simulink model "QD2_Sim_Dual"  (R2023b)
settings: Solver=FixedStepDiscrete  StartTime=0.0  StopTime=400  FixedStep=0.002  RelTol=1e-3
PreLoadFcn:
  | % QD2_Sim_Dual: agrega lib/ y sim/ al path antes de cargar (enlaces a QD2_Mission_Lib)
  | qd2_c = {pwd};
  | qd2_w = which('QD2_Sim_Dual');
  | if ~isempty(qd2_w), qd2_c{end+1} = fileparts(qd2_w); end
  | for qd2_i = 1:numel(qd2_c)
  |     qd2_d = qd2_c{qd2_i};
  |     for qd2_k = 1:4
  |         if exist(fullfile(qd2_d, 'lib', 'QD2_Mission_Lib.slx'), 'file')
  |             addpath(fullfile(qd2_d, 'lib'));
  |             addpath(fullfile(qd2_d, 'sim'));
  |             break;
  |         end
  |         qd2_d = fileparts(qd2_d);
  |     end
  | end
  | clear qd2_c qd2_w qd2_i qd2_d qd2_k
PostLoadFcn:
  | % QD2_Sim_Dual: rutas de lib/ (funciones qd2_* y QD2_Mission_Lib) y sim/
  | qd2_d = fileparts(get_param(bdroot, 'FileName'));
  | for qd2_k = 1:4
  |     if exist(fullfile(qd2_d, 'lib', 'qd2_params.m'), 'file'), break; end
  |     qd2_d = fileparts(qd2_d);
  | end
  | addpath(fullfile(qd2_d, 'lib'));
  | addpath(fullfile(qd2_d, 'sim'));
  | clear qd2_d qd2_k
InitFcn:
  | % QD2_Sim_Dual: rutas de lib/ (funciones qd2_* y QD2_Mission_Lib) y sim/
  | qd2_d = fileparts(get_param(bdroot, 'FileName'));
  | for qd2_k = 1:4
  |     if exist(fullfile(qd2_d, 'lib', 'qd2_params.m'), 'file'), break; end
  |     qd2_d = fileparts(qd2_d);
  | end
  | addpath(fullfile(qd2_d, 'lib'));
  | addpath(fullfile(qd2_d, 'sim'));
  | clear qd2_d qd2_k
  | % Parámetros (config/estacion.json es la única fuente de verdad)
  | QD2P = qd2_params_from_config();
  | QD2_SIM = qd2_sim_parametros();
  | % La versión la fija el bloque constante VERSION de la raíz
  | QD2_VERSION = str2double(get_param([bdroot '/' sprintf('VERSION\n(1 = PID, 2 = MPC)')], 'Value'));
libraries: simulink x1
(part 2 of 2)

== matlab function QD2_Sim_Dual/MISSION SUPERVISOR/MATLAB Function ==
  data: t input; sp1 output size=[4 1]; pose1 input; pose2 input; trk input; py input; ab input; sp2 output size=[4 1]; ctx output size=[7 1]; info output size=[40 1]; estado output size=1; cmd1 output size=[3 1]; cmd2 output size=[3 1]; P parameter; version parameter
function [sp1, sp2, ctx, info, estado, cmd1, cmd2] = fcn(t, pose1, pose2, trk, py, ab, P, version)
%#codegen
% MISSION SUPERVISOR: qd2_mission_step (FSM de ARQUITECTURA §3.3) para los 2 drones.
% ab = Onboard Status [fsm1 fsm2 cod1 cod2] (MPC LINK CHECK; fsm 0 = desconocida;
% cod 0 bien, 1 protocolo MPC incorrecto, 2 enlace perdido).
persistent s
if isempty(s)
    s = qd2_mission_init(P);
end
in.t = t;
in.pose1 = [pose1(1) pose1(2) pose1(3) pose1(4)];
in.pose2 = [pose2(1) pose2(2) pose2(3) pose2(4)];
in.tracked1 = trk(1);
in.tracked2 = trk(2);
in.py = py(:);
in.version = version;
in.fsm_a_bordo = [ab(1) ab(2)];
in.proto_mal = [ab(3) ab(4)];
[s, ~, ~, tel] = qd2_mission_step(s, in, P);
sp1 = [tel.sp1(1); tel.sp1(2); tel.sp1(3); tel.sp1(4)];
sp2 = [tel.sp2(1); tel.sp2(2); tel.sp2(3); tel.sp2(4)];
cmd1 = [tel.arm(1); tel.takeoff(1); tel.estop(1)];
cmd2 = [tel.arm(2); tel.takeoff(2); tel.estop(2)];
ctx = zeros(7, 1);
ctx(1) = tel.explorer_id;
for k = 1:6
    ctx(k+1) = tel.ctx_guard(k);
end
% Mission Info [40] (orden fijo, lo leen el TELEMETRY PACK, el OPERATOR SAFETY LAYER
% (info(1)) y el SETPOINT RATE LIMITER (info(38:39)))
info = zeros(40, 1);
info(1) = tel.mission_state;      info(2) = tel.explorer_id;
info(3) = tel.responder_id;       info(4) = tel.explorer_wp_idx;
info(5) = tel.explorer_wp_total;  info(6) = tel.responder_target_id;
info(7) = tel.n_targets_known;    info(8) = tel.n_targets_visited;
info(9) = tel.explorer_done;      info(10) = tel.visited_mask;
info(11) = tel.marking_progress;  info(12) = tel.queue_length;
info(13) = tel.cmd_seq_ack;
info(14) = tel.home1(1);  info(15) = tel.home1(2);
info(16) = tel.home2(1);  info(17) = tel.home2(2);
info(18) = tel.role1;     info(19) = tel.role2;
info(20) = tel.alerta;    info(21) = tel.home_ok;
info(22) = tel.pausa_por_trk;  info(23) = tel.hb_ok;
info(24) = tel.pausa_por_hb;   info(25) = tel.z_E;
info(26) = tel.z_R;       info(27) = tel.d_min_h;
info(28) = tel.t_mark;    info(29) = tel.r_marking;
% falla a bordo por dron (0, 9, 10), fase de la reacción, objetivo rotando y(56:60)
info(30) = tel.falla(1);  info(31) = tel.falla(2);
info(32) = tel.falla_fase;
for k = 1:5
    info(32 + k) = tel.obj_rot(k);
end
% 1 = el dron se aparta de un dron en falla (límite xy P.falla_rate_xy)
info(38) = tel.escape(1); info(39) = tel.escape(2);
estado = tel.mission_state;

== matlab function QD2_Sim_Dual/MPC LINK CHECK/MATLAB Function ==
  data: t input; est output size=[4 1]; tel1 input; tel2 input; lb1 input; lb2 input; cs1 input; cs2 input; P parameter; version parameter
function est = fcn(t, tel1, tel2, lb1, lb2, cs1, cs2, P, version)
%#codegen
% MPC LINK CHECK (qd2_enlace_mpc): valida la respuesta de 8 doubles de cada dron
% (§3.2: y(8) = 2, FSM entera 1..9). est = [fsm1 fsm2 cod1 cod2]
% (cod 0 bien, 1 protocolo incorrecto sostenido, 2 enlace perdido).
persistent tm
if isempty(tm)
    tm = [-1 -1 0 0];
end
y1 = zeros(1, 8);
y2 = zeros(1, 8);
for k = 1:8
    y1(k) = tel1(k);
    y2(k) = tel2(k);
end
[e, tm] = qd2_enlace_mpc(tm, t, y1, y2, [lb1(1) lb2(1)], [cs1(1) cs2(1)], P, version);
est = [e(1); e(2); e(3); e(4)];

== matlab function QD2_Sim_Dual/QDRONE 2 #1 (SIM)/PLANT (qd2_quad_plant) ==
  data: u input; x output size=[10 1]; F input; home input; QD2P parameter
function x = fcn(u, F, home, QD2P)
%#codegen
% PLANTA: qd2_quad_plant (traslación 3D, actitud y empuje de 1er orden, suelo).
persistent xs
if isempty(xs)
    xs = zeros(10, 1);
    xs(1) = home(1);
    xs(2) = home(2);
end
xs = qd2_quad_plant(xs, u, F, 0.002, QD2P.planta);
x = xs;

== matlab function QD2_Sim_Dual/OPERATOR SAFETY LAYER/MATLAB Function ==
  data: t input; trig1 output size=[1 4]; sw input; cmd1 input; cmd2 input; modo_sel input; trig2 output size=[1 4]; modo_ef output size=1
function [trig1, trig2, modo_ef] = fcn(t, sw, cmd1, cmd2, modo_sel)
%#codegen
% OPERATOR SAFETY LAYER (versión simple, interfaz de la simulación QD2_Sim_Dual).
% sw = [Arm Takeoff EStop 0]. modo 0 = MISIÓN, 1 = MANUAL Equipo2 (solo dron 1).
EXT = false;
D_MIN = 0.9;
estado = -1;
fsm = [0 0];
d1 = zeros(7, 1);
d2 = zeros(7, 1);
T_ARM_MIN = 1.0;    % s armado antes de permitir takeoff (a bordo: trigger_2 en IDLE = Error)
T_ACEPTA = 2.0;     % s para que el supervisor acepte el LAND ALL del operador
T_RESPALDO = 90.0;  % s máximos con Takeoff/Land abajo antes del aterrizaje crudo
Z_SUELO = 0.10;     % m
persistent modo t_arm a_prev to_prev sw_prev t_bajo n_req lat_to lat_arm
if isempty(modo)
    modo = double(modo_sel > 0.5);
    t_arm = [-1 -1];
    a_prev = [0 0];
    to_prev = [0 0];
    sw_prev = [double(sw(1) > 0.5) double(sw(2) > 0.5) double(sw(3) > 0.5)];
    t_bajo = -1;
    n_req = 0;
    lat_to = 0;
    lat_arm = 0;
end
sw_arm = sw(1) > 0.5;
sw_to = sw(2) > 0.5;
sw_es = sw(3) > 0.5;
z = [d1(3) d2(3)];
rastreo = [d1(7) > 0.5 && isfinite(d1(3)), d2(7) > 0.5 && isfinite(d2(3))];
armado = a_prev(1) > 0.5 || a_prev(2) > 0.5;
volando = to_prev(1) > 0.5 || to_prev(2) > 0.5;

% ---- Cambio de modo: SOLO en tierra, con los dos Flight State en Idle (0),
% los dos desarmados y los switches Arm y Takeoff ABAJO. Así un cambio del
% selector hecho en vuelo queda pendiente y nunca dispara arm/takeoff solo:
% el operador tiene que bajar los switches y volver a subirlos.
sel = double(modo_sel > 0.5);
suelo = true;
for i = 1:2
    if rastreo(i) && z(i) >= Z_SUELO
        suelo = false;
    end
end
if sel ~= modo && fsm(1) == 0 && fsm(2) == 0 && ~armado && ~volando && ~sw_arm && ~sw_to && suelo
    modo = sel;
    t_arm = [-1 -1];
end

% ---- Peticiones del operador en modo MISIÓN (flancos de los switches)
if EXT && modo < 0.5
    if sw_prev(2) > 0.5 && ~sw_to && (armado || volando)
        n_req = n_req + 1;      % Takeoff/Land abajo -> LAND ALL ordenado
        lat_to = 1;
        t_bajo = t;
    end
    if sw_prev(1) > 0.5 && ~sw_arm && armado
        n_req = n_req + 1;      % Arm abajo (corte, como el original) -> LAND ALL
        lat_arm = 1;
    end
    if sw_prev(3) < 0.5 && sw_es && armado
        n_req = n_req + 1;      % E-stop -> LAND ALL (la misión no sigue)
    end
end
if sw_to
    lat_to = 0;
    t_bajo = -1;
end
if sw_arm
    lat_arm = 0;
end
sw_prev = [double(sw_arm) double(sw_to) double(sw_es)];

% ---- Disparos pedidos
if modo > 0.5
    a = [double(sw_arm) 0];
    to_req = [sw_to false];
    es = [double(sw_es) double(sw_es)];
else
    a = [double(sw_arm && cmd1(1) > 0.5), double(sw_arm && cmd2(1) > 0.5)];
    es = [double(sw_es || cmd1(3) > 0.5), double(sw_es || cmd2(3) > 0.5)];
    if EXT
        % Takeoff/Land = PERMISO para despegar. En vuelo, bajarlo NO corta el
        % takeoff de golpe (cada dron aterrizaría en su x,y: E caería sobre R
        % en la versión MPC); pide LAND ALL y el takeoff sigue al supervisor.
        to_req = [cmd1(2) > 0.5 && (sw_to || to_prev(1) > 0.5), ...
                  cmd2(2) > 0.5 && (sw_to || to_prev(2) > 0.5)];
    else
        to_req = [sw_to && cmd1(2) > 0.5, sw_to && cmd2(2) > 0.5];
    end
end

% ---- Respaldo crudo: el supervisor no aceptó el LAND ALL (estado distinto de
% LANDING/DONE/en tierra) en T_ACEPTA, o pasaron T_RESPALDO con Takeoff abajo.
% Suelta el takeoff, pero NUNCA el de un dron que tiene al otro DEBAJO a
% menos de d_min_h en horizontal (aterrizaría encima / en su downwash).
respaldo = 0;
if EXT && modo < 0.5 && t_bajo >= 0 && volando
    acepto = (estado == 7) || (estado == 8) || (estado <= 2);
    if (~acepto && (t - t_bajo) >= T_ACEPTA) || ((t - t_bajo) >= T_RESPALDO)
        respaldo = 1;
        dh = sqrt((d1(1) - d2(1))^2 + (d1(2) - d2(2))^2);
        for i = 1:2
            o = 3 - i;
            debajo = rastreo(o) && rastreo(i) && dh < D_MIN && z(o) < z(i) - 0.15;
            if ~debajo
                to_req(i) = false;
            end
        end
    end
end

% ---- Takeoff efectivo: >= T_ARM_MIN después de armar (también en MANUAL).
to = [0 0];
for i = 1:2
    if a(i) > 0.5
        if t_arm(i) < 0
            t_arm(i) = t;
        end
    else
        t_arm(i) = -1;
    end
    if modo > 0.5
        % manual: igual que el original una vez en vuelo (el takeoff sigue al
        % switch aunque se baje Arm); para despegar exige 1 s armado
        if to_req(i) && (to_prev(i) > 0.5 || (a(i) > 0.5 && (t - t_arm(i)) >= T_ARM_MIN))
            to(i) = 1;
        end
    elseif to_req(i) && a(i) > 0.5 && (t - t_arm(i)) >= T_ARM_MIN
        to(i) = 1;
    end
end

% ---- Alerta del operador para la telemetría (y(55))
codigo = 0;
if sw_es
    codigo = 5;
elseif respaldo > 0.5
    codigo = 8;
elseif lat_arm > 0.5
    codigo = 7;
elseif lat_to > 0.5
    codigo = 6;
end
a_prev = a;
to_prev = to;
trig1 = [a(1) to(1) es(1) 0];
trig2 = [a(2) to(2) es(2) 0];
modo_ef = modo;

== matlab function QD2_Sim_Dual/ROLE & HOME ASSIGNMENT/MATLAB Function ==
  data: d1 input; pose1 output size=[4 1]; d2 input; pose2 output size=[4 1]; trk output size=[2 1]; prev output size=[8 1]; P parameter; version parameter
function [pose1, pose2, trk, prev] = fcn(d1, d2, P, version)
%#codegen
% ROLE & HOME ASSIGNMENT. d1/d2 = Corrected Pose Data [x y z roll pitch yaw isTracking].
% prev = [explorer_id responder_id home1x home1y home2x home2y d_homes start_ok] (vista previa;
% el MISSION SUPERVISOR fija roles y homes con START).
pose1 = [d1(1); d1(2); d1(3); d1(6)];
pose2 = [d2(1); d2(2); d2(3); d2(6)];
trk = [d1(7); d2(7)];
[e, r, h1, h2, ok] = qd2_assign_roles(pose1, pose2, trk(1), trk(2));
dh = sqrt((h1(1) - h2(1))^2 + (h1(2) - h2(2))^2);
if version > 1.5
    umbral = P.d_home_min_mpc;
else
    umbral = P.d_min_h + P.guard_margen;
end
prev = [e; r; h1(1); h1(2); h2(1); h2(2); dh; double(ok > 0.5 && dh >= umbral)];

== matlab function QD2_Sim_Dual/SEPARATION GUARD/MATLAB Function ==
  data: pose1 input; sp1o output size=[4 1]; pose2 input; sp1 input; sp2 input; ctx input; sp2o output size=[4 1]; activo output size=1; P parameter
function [sp1o, sp2o, activo] = fcn(pose1, pose2, sp1, sp2, ctx, P)
%#codegen
% SEPARATION GUARD (versión PID): qd2_separation_guard por rol.
persistent gs eid_prev
if isempty(gs)
    gs = qd2_guard_init();
    eid_prev = ctx(1);
end
if ctx(1) ~= eid_prev
    gs = qd2_guard_init();   % los roles cambiaron: el estado ya no aplica
    eid_prev = ctx(1);
end
c6 = [ctx(2) ctx(3) ctx(4) ctx(5) ctx(6) ctx(7)];
p1 = [pose1(1) pose1(2) pose1(3)];
p2 = [pose2(1) pose2(2) pose2(3)];
s1 = [sp1(1) sp1(2) sp1(3) sp1(4)];
s2 = [sp2(1) sp2(2) sp2(3) sp2(4)];
if ctx(1) == 2
    [eO, rO, act, gs] = qd2_separation_guard(p2, p1, s2, s1, P, gs, c6);
    sp1o = [rO(1); rO(2); rO(3); rO(4)];
    sp2o = [eO(1); eO(2); eO(3); eO(4)];
else
    [eO, rO, act, gs] = qd2_separation_guard(p1, p2, s1, s2, P, gs, c6);
    sp1o = [eO(1); eO(2); eO(3); eO(4)];
    sp2o = [rO(1); rO(2); rO(3); rO(4)];
end
activo = double(act);

== matlab function QD2_Sim_Dual/SETPOINT RATE LIMITER QDrone 1/MATLAB Function ==
  data: t input; u input; y output size=[1 4]; trig input; info input; P parameter; dron parameter
function y = fcn(t, u, trig, info, P, dron)
%#codegen
% SETPOINT RATE LIMITER: limita x,y por norma (camino recto), z y yaw por eje.
% info(37 + dron) = 1: el dron se aparta de un dron en falla -> límite xy P.falla_rate_xy.
persistent yp tp
uu = [u(1); u(2); u(3); u(4)];
if isempty(yp)
    yp = uu;
    tp = t;
end
dt = t - tp;
if dt < 0
    dt = 0;
end
tp = t;
if ~all(isfinite(uu))
    uu = yp;
end
if trig(1) < 0.5
    yp = uu;   % desarmado: sigue la consigna del supervisor sin limitar
else
    rate = [P.pid.rate_xy; P.pid.rate_xy; P.pid.rate_z; P.pid.rate_yaw];
    ie = min(max(round(37 + dron), 38), 39);
    if info(ie) > 0.5
        rate(1) = P.falla_rate_xy;
        rate(2) = P.falla_rate_xy;
    end
    yp = qd2_rate_limit(yp, uu, rate, dt, 1);
end
% fila [1x4], igual que la salida del Rate Limiter2 original
y = [yp(1) yp(2) yp(3) yp(4)];

== matlab function QD2_Sim_Dual/SETPOINT RATE LIMITER QDrone 2/MATLAB Function ==
  data: t input; u input; y output size=[1 4]; trig input; info input; P parameter; dron parameter
function y = fcn(t, u, trig, info, P, dron)
%#codegen
% SETPOINT RATE LIMITER: limita x,y por norma (camino recto), z y yaw por eje.
% info(37 + dron) = 1: el dron se aparta de un dron en falla -> límite xy P.falla_rate_xy.
persistent yp tp
uu = [u(1); u(2); u(3); u(4)];
if isempty(yp)
    yp = uu;
    tp = t;
end
dt = t - tp;
if dt < 0
    dt = 0;
end
tp = t;
if ~all(isfinite(uu))
    uu = yp;
end
if trig(1) < 0.5
    yp = uu;   % desarmado: sigue la consigna del supervisor sin limitar
else
    rate = [P.pid.rate_xy; P.pid.rate_xy; P.pid.rate_z; P.pid.rate_yaw];
    ie = min(max(round(37 + dron), 38), 39);
    if info(ie) > 0.5
        rate(1) = P.falla_rate_xy;
        rate(2) = P.falla_rate_xy;
    end
    yp = qd2_rate_limit(yp, uu, rate, dt, 1);
end
% fila [1x4], igual que la salida del Rate Limiter2 original
y = [yp(1) yp(2) yp(3) yp(4)];

== matlab function QD2_Sim_Dual/STACKING INFO/MATLAB Function ==
  data: d1 input; x1 output size=[1 8]; d2 input; v1 input; v2 input; modo input; x2 output size=[1 8]; dz output size=1
function [x1, x2, dz] = fcn(d1, d2, v1, v2, modo)
%#codegen
% STACKING INFO (versión MPC): estado del OTRO dron para el MPC a bordo (§3.2, índices 17-24):
% [x y z vx vy vz del otro, mpc_mode, 2].
x1 = zeros(1, 8);
x2 = zeros(1, 8);
if d2(7) > 0.5
    x1(1:3) = [d2(1); d2(2); d2(3)];
    x1(4:6) = [v2(1); v2(2); v2(3)];
else
    x1(1:6) = NaN;
end
if d1(7) > 0.5
    x2(1:3) = [d1(1); d1(2); d1(3)];
    x2(4:6) = [v1(1); v1(2); v1(3)];
else
    x2(1:6) = NaN;
end
x1(7) = modo;
x2(7) = modo;
% índice 24 = 2: etiqueta "protocolo MPC v1" (el PROTOCOL CHECK a bordo solo acepta 2)
x1(8) = 2;
x2(8) = 2;
dz = d1(3) - d2(3);

== matlab function QD2_Sim_Dual/TELEMETRY PACK/MATLAB Function ==
  data: t input; y output size=[64 1]; info input; guard input; d1 input; d2 input; des1 input; des2 input; v1 input; v2 input; st input; version parameter
function y = fcn(t, info, guard, d1, d2, des1, des2, v1, v2, st, version)
%#codegen
% TELEMETRY PACK: 64 doubles Simulink -> Python (ARQUITECTURA §3.3) con qd2_telemetry_pack.
tel.mission_state = info(1);
tel.explorer_id = info(2);
tel.responder_id = info(3);
tel.explorer_wp_idx = info(4);
tel.explorer_wp_total = info(5);
tel.responder_target_id = info(6);
tel.n_targets_known = info(7);
tel.n_targets_visited = info(8);
tel.explorer_done = info(9);
tel.visited_mask = info(10);
tel.marking_progress = info(11);
tel.queue_length = info(12);
tel.cmd_seq_ack = info(13);
tel.home1 = [info(14) info(15)];
tel.home2 = [info(16) info(17)];
tel.role1 = info(18);
tel.role2 = info(19);
% y(56:60): objetivo de la tabla que toca en este mensaje [id clase x y estado]
tel.obj_rot = [info(33) info(34) info(35) info(36) info(37)];
% alerta: la del operador (Drone Status(10): 5 E-stop, 6 Takeoff abajo, 7 Arm abajo,
% 8 respaldo crudo) tiene prioridad sobre la del supervisor (0-4, 9 falla a bordo,
% 10 protocolo MPC incorrecto)
alerta = info(20);
if numel(st) >= 10
    ov = st(min(10, numel(st)));
    if ov > 0.5
        alerta = ov;
    end
end
tel.alerta = alerta;
pose1 = [d1(1); d1(2); d1(3); d1(6)];
pose2 = [d2(1); d2(2); d2(3); d2(6)];
% comm_ok = sin Communication Issue y loopback < 0.5 s
comm1 = double(st(5) < 0.5 && st(7) < 0.5);
comm2 = double(st(6) < 0.5 && st(8) < 0.5);
aux = [d1(7) d2(7) st(1) st(2) st(3) st(4) comm1 comm2];
% y(61:63): roll y pitch (rad) de la misma Corrected Pose Data [x y z roll pitch yaw trk];
% qd2_telemetry_pack elige los del explorador y pone y(63) = 1 si son válidos
att = [d1(4) d1(5) d2(4) d2(5)];
y = qd2_telemetry_pack(t, tel, version, guard, pose1, pose2, ...
    [des1(1) des1(2) des1(3) des1(4)], [des2(1) des2(2) des2(3) des2(4)], ...
    [v1(1) v1(2) v1(3)], [v2(1) v2(2) v2(3)], aux, att);

== matlab function QD2_Sim_Dual/QDRONE 2 #1 (SIM)/ON-BOARD STACK (FSM + PIV or MPC) ==
  data: trig input; u output size=[4 1]; des input; mpcx input; x input; version input; dpose input; t input; st output size=[5 1]; QD2P parameter; QD2_SIM parameter
function [u, st] = fcn(trig, des, mpcx, x, version, dpose, t, QD2P, QD2_SIM)
%#codegen
% STACK A BORDO SIMULADO del QDrone 2 #1 (500 Hz): FSM + PIV original o MPC
% (qd2_onboard_step), con la estimación y los errores del stack real.
% trig = [arm takeoff estop 0], des = pose deseada [x y z yaw],
% mpcx = [otro dron x y z vx vy vz, mpc_mode, 0] (índices 17-24 del paquete MPC),
% x = estado verdadero de la planta (solo para la IMU: roll, pitch, aceleración),
% dpose = OptiTrack [x y z roll pitch yaw isTracking] (100 Hz, NaN sin rastreo).
ID = 1;
NB = 64;
persistent ob bat buf kb pos vf1 vf2 vest vprev pprev t_trk t_com paq T7 u_prev fh t_ap
dt = 0.002;
if isempty(ob)
    ob = qd2_onboard_init(QD2P);
    bat = 16.4;
    buf = zeros(7, NB);
    for j = 1:NB
        buf(:, j) = [x(1); x(2); x(3); x(7); x(8); x(9); 1];
    end
    kb = 1;
    pos = [x(1); x(2); x(3); x(9)];
    pprev = pos(1:3);
    vf1 = zeros(3, 1); vf2 = zeros(3, 1); vest = zeros(3, 1);
    vprev = [x(4); x(5); x(6)];
    t_trk = 0; t_com = 0; T7 = 0;
    paq = [trig(:); des(:); mpcx(:); dpose(:)];
    u_prev = zeros(4, 1);
    fh = false; t_ap = 0;
end
% ---- enlace PC -> dron: pérdidas programadas QD2_SIM.comm_off [dron t1 t2] ----
sin_enlace = false;
co = QD2_SIM.comm_off;
for k = 1:size(co, 1)
    if co(k,1) == ID && t >= co(k,2) && t < co(k,3)
        sin_enlace = true;
    end
end
if ~sin_enlace
    paq = [trig(:); des(:); mpcx(:); dpose(:)];   % "most recent": sin enlace queda el último
    t_com = 0;
else
    t_com = t_com + dt;
end
tr = paq(1:4); ds = paq(5:8); mx = paq(9:16); dp = paq(17:23);
% ---- estimación a bordo ------------------------------------------------
% pose OptiTrack con latencia (buffer circular a 500 Hz)
buf(:, kb) = dp;
nl = min(max(round(QD2_SIM.lat_pose/dt), 0), NB - 1);
j = kb - nl;
if j < 1, j = j + NB; end
dd = buf(:, j);
kb = kb + 1;
if kb > NB, kb = 1; end
trk = dd(7) > 0.5 && all(isfinite(dd(1:6)));
if trk
    pos = [dd(1); dd(2); dd(3); dd(6)];
end
if QD2_SIM.pose_onboard < 0.5
    pos = [x(1); x(2); x(3); x(9)];   % estimación ideal (solo para comparar)
    trk = true;
end
% velocidad: complementario acelerómetro + derivada de OptiTrack (LPF 2o orden
% wn = 50 rad/s, zeta = 1; Kp3 = 4), como HORIZON FRAME CONVERSION AND ESTIMATION
dpos = (pos(1:3) - pprev)/dt;
pprev = pos(1:3);
a = 50*dt;
vf1 = vf1 + a*(dpos - vf1);
vf2 = vf2 + a*(vf1 - vf2);
acc = ([x(4); x(5); x(6)] - vprev)/dt;
vprev = [x(4); x(5); x(6)];
vest = vest + dt*(acc + 4*(vf2 - vest));
if QD2_SIM.pose_onboard < 0.5
    vest = [x(4); x(5); x(6)];
end
x_est = [pos(1); pos(2); pos(3); vest(1); vest(2); vest(3); x(7); x(8); pos(4)];
% ---- errores del stack original (STATE MACHINE SIGNALS) ----------------
if ~trk && t > 1
    t_trk = t_trk + dt;
else
    t_trk = 0;
end
err_trk = t_trk >= 0.2;
err_com = t > 3 && t_com >= 0.5;
if (err_trk || err_com) && ob.fsm <= 6
    ob.fsm = 7;                % Error -> EMERGENCY STOP (rampa)
    T7 = u_prev(1);
end
if t_com >= 1.0 && tr(1) > 0.5 && ob.fsm ~= 9
    ob.fsm = 9;                % FLIGHT SAFETY: enlace perdido 1 s y armado -> corta motores
end
% ---- falla a bordo programada (QD2_SIM.falla_fsm [dron t]) o al estar apilados
% (QD2_SIM.falla_apilado: 1 = falla el de ARRIBA, 2 = el de ABAJO, tras 1 s con
% dh < 0.15 m y dz > 0.5 m): Error -> estado 7 como el stack original
falla = false;
fa = QD2_SIM.falla_fsm;
for k = 1:size(fa, 1)
    if fa(k,1) == ID && fa(k,2) >= 0 && t >= fa(k,2)
        falla = true;
    end
end
if QD2_SIM.falla_apilado > 0.5 && all(isfinite(mx(1:3)))
    dz = x(3) - mx(3);
    apil = sqrt((x(1) - mx(1))^2 + (x(2) - mx(2))^2) < 0.15 && abs(dz) > 0.5 && min(x(3), mx(3)) > 0.2;
    yo_arriba = dz > 0;
    if apil && ((QD2_SIM.falla_apilado < 1.5 && yo_arriba) || (QD2_SIM.falla_apilado > 1.5 && ~yo_arriba))
        t_ap = t_ap + dt;
    else
        t_ap = 0;
    end
    if t_ap >= 1.0
        falla = true;
    end
end
if falla && ~fh && ob.fsm >= 1 && ob.fsm <= 6
    fh = true;
    ob.fsm = 7;
    T7 = u_prev(1);
end
if tr(3) > 0.5
    ob.fsm = 9;                % E-stop: corte de motores (estado 8 -> 9 del original)
end
modo = 1;
if version > 1.5 && mx(7) > 0.5
    modo = 2;
end
otro = [mx(1); mx(2); mx(3); mx(4); mx(5); mx(6)];
ref = [ds(1) ds(2) ds(3) ds(4)];
if ob.fsm == 7
    % actitud nivelada, sin control de posición, empuje baja a 1.75 N/s
    T7 = max(T7 - 1.75*dt, 0);
    u = [T7; 0; 0; 0];
    if T7 <= 7.38
        ob.fsm = 9;
        u = zeros(4, 1);
    end
else
    [u, ob] = qd2_onboard_step(ob, tr(1), tr(2), ref, x_est, otro, QD2P, dt, modo);
end
u_prev = u;
bat = bat - dt*3.2e-4*u(1);   % descarga simple: ~0.005 V/s en hover
est = 3;
if ob.fsm >= 4 && ob.fsm <= 6
    if modo > 1.5
        est = ob.status;
    else
        est = 4;
    end
end
st = [ob.fsm; bat; est; u(1); double(err_com)];

== matlab function QD2_Sim_Dual/VELOCITY ESTIMATE QDrone 1/MATLAB Function ==
  data: t input; v output size=[3 1]; d input
function v = fcn(t, d)
%#codegen
% VELOCITY ESTIMATE: derivada entre muestras nuevas de OptiTrack + filtro de 1er orden.
TAU = 0.04;
persistent pl tl vt vf tp
x = [d(1); d(2); d(3)];
if isempty(pl)
    pl = x;
    tl = t - 1;
    vt = zeros(3, 1);
    vf = zeros(3, 1);
    tp = t;
end
dtp = t - tp;
if dtp < 0
    dtp = 0;
end
tp = t;
if all(isfinite(x)) && d(7) > 0.5
    if any(x ~= pl)
        dtm = t - tl;
        if dtm > 1e-4 && dtm < 0.5
            vt = (x - pl)/dtm;
        else
            vt = zeros(3, 1);
        end
        pl = x;
        tl = t;
    elseif t - tl > 0.05
        vt = zeros(3, 1);
    end
else
    vt = zeros(3, 1);
    tl = t - 1;
end
a = dtp/(TAU + dtp);
vf = vf + a*(vt - vf);
v = vf;

== matlab function QD2_Sim_Dual/VELOCITY ESTIMATE QDrone 2/MATLAB Function ==
  data: t input; v output size=[3 1]; d input
function v = fcn(t, d)
%#codegen
% VELOCITY ESTIMATE: derivada entre muestras nuevas de OptiTrack + filtro de 1er orden.
TAU = 0.04;
persistent pl tl vt vf tp
x = [d(1); d(2); d(3)];
if isempty(pl)
    pl = x;
    tl = t - 1;
    vt = zeros(3, 1);
    vf = zeros(3, 1);
    tp = t;
end
dtp = t - tp;
if dtp < 0
    dtp = 0;
end
tp = t;
if all(isfinite(x)) && d(7) > 0.5
    if any(x ~= pl)
        dtm = t - tl;
        if dtm > 1e-4 && dtm < 0.5
            vt = (x - pl)/dtm;
        else
            vt = zeros(3, 1);
        end
        pl = x;
        tl = t;
    elseif t - tl > 0.05
        vt = zeros(3, 1);
    end
else
    vt = zeros(3, 1);
    tl = t - 1;
end
a = dtp/(TAU + dtp);
vf = vf + a*(vt - vf);
v = vf;

== matlab function QD2_Sim_Dual/QDRONE 2 #2 (SIM)/ON-BOARD STACK (FSM + PIV or MPC) ==
  data: trig input; u output size=[4 1]; des input; mpcx input; x input; version input; dpose input; t input; st output size=[5 1]; QD2P parameter; QD2_SIM parameter
function [u, st] = fcn(trig, des, mpcx, x, version, dpose, t, QD2P, QD2_SIM)
%#codegen
% STACK A BORDO SIMULADO del QDrone 2 #2 (500 Hz): FSM + PIV original o MPC
% (qd2_onboard_step), con la estimación y los errores del stack real.
% trig = [arm takeoff estop 0], des = pose deseada [x y z yaw],
% mpcx = [otro dron x y z vx vy vz, mpc_mode, 0] (índices 17-24 del paquete MPC),
% x = estado verdadero de la planta (solo para la IMU: roll, pitch, aceleración),
% dpose = OptiTrack [x y z roll pitch yaw isTracking] (100 Hz, NaN sin rastreo).
ID = 2;
NB = 64;
persistent ob bat buf kb pos vf1 vf2 vest vprev pprev t_trk t_com paq T7 u_prev fh t_ap
dt = 0.002;
if isempty(ob)
    ob = qd2_onboard_init(QD2P);
    bat = 16.4;
    buf = zeros(7, NB);
    for j = 1:NB
        buf(:, j) = [x(1); x(2); x(3); x(7); x(8); x(9); 1];
    end
    kb = 1;
    pos = [x(1); x(2); x(3); x(9)];
    pprev = pos(1:3);
    vf1 = zeros(3, 1); vf2 = zeros(3, 1); vest = zeros(3, 1);
    vprev = [x(4); x(5); x(6)];
    t_trk = 0; t_com = 0; T7 = 0;
    paq = [trig(:); des(:); mpcx(:); dpose(:)];
    u_prev = zeros(4, 1);
    fh = false; t_ap = 0;
end
% ---- enlace PC -> dron: pérdidas programadas QD2_SIM.comm_off [dron t1 t2] ----
sin_enlace = false;
co = QD2_SIM.comm_off;
for k = 1:size(co, 1)
    if co(k,1) == ID && t >= co(k,2) && t < co(k,3)
        sin_enlace = true;
    end
end
if ~sin_enlace
    paq = [trig(:); des(:); mpcx(:); dpose(:)];   % "most recent": sin enlace queda el último
    t_com = 0;
else
    t_com = t_com + dt;
end
tr = paq(1:4); ds = paq(5:8); mx = paq(9:16); dp = paq(17:23);
% ---- estimación a bordo ------------------------------------------------
% pose OptiTrack con latencia (buffer circular a 500 Hz)
buf(:, kb) = dp;
nl = min(max(round(QD2_SIM.lat_pose/dt), 0), NB - 1);
j = kb - nl;
if j < 1, j = j + NB; end
dd = buf(:, j);
kb = kb + 1;
if kb > NB, kb = 1; end
trk = dd(7) > 0.5 && all(isfinite(dd(1:6)));
if trk
    pos = [dd(1); dd(2); dd(3); dd(6)];
end
if QD2_SIM.pose_onboard < 0.5
    pos = [x(1); x(2); x(3); x(9)];   % estimación ideal (solo para comparar)
    trk = true;
end
% velocidad: complementario acelerómetro + derivada de OptiTrack (LPF 2o orden
% wn = 50 rad/s, zeta = 1; Kp3 = 4), como HORIZON FRAME CONVERSION AND ESTIMATION
dpos = (pos(1:3) - pprev)/dt;
pprev = pos(1:3);
a = 50*dt;
vf1 = vf1 + a*(dpos - vf1);
vf2 = vf2 + a*(vf1 - vf2);
acc = ([x(4); x(5); x(6)] - vprev)/dt;
vprev = [x(4); x(5); x(6)];
vest = vest + dt*(acc + 4*(vf2 - vest));
if QD2_SIM.pose_onboard < 0.5
    vest = [x(4); x(5); x(6)];
end
x_est = [pos(1); pos(2); pos(3); vest(1); vest(2); vest(3); x(7); x(8); pos(4)];
% ---- errores del stack original (STATE MACHINE SIGNALS) ----------------
if ~trk && t > 1
    t_trk = t_trk + dt;
else
    t_trk = 0;
end
err_trk = t_trk >= 0.2;
err_com = t > 3 && t_com >= 0.5;
if (err_trk || err_com) && ob.fsm <= 6
    ob.fsm = 7;                % Error -> EMERGENCY STOP (rampa)
    T7 = u_prev(1);
end
if t_com >= 1.0 && tr(1) > 0.5 && ob.fsm ~= 9
    ob.fsm = 9;                % FLIGHT SAFETY: enlace perdido 1 s y armado -> corta motores
end
% ---- falla a bordo programada (QD2_SIM.falla_fsm [dron t]) o al estar apilados
% (QD2_SIM.falla_apilado: 1 = falla el de ARRIBA, 2 = el de ABAJO, tras 1 s con
% dh < 0.15 m y dz > 0.5 m): Error -> estado 7 como el stack original
falla = false;
fa = QD2_SIM.falla_fsm;
for k = 1:size(fa, 1)
    if fa(k,1) == ID && fa(k,2) >= 0 && t >= fa(k,2)
        falla = true;
    end
end
if QD2_SIM.falla_apilado > 0.5 && all(isfinite(mx(1:3)))
    dz = x(3) - mx(3);
    apil = sqrt((x(1) - mx(1))^2 + (x(2) - mx(2))^2) < 0.15 && abs(dz) > 0.5 && min(x(3), mx(3)) > 0.2;
    yo_arriba = dz > 0;
    if apil && ((QD2_SIM.falla_apilado < 1.5 && yo_arriba) || (QD2_SIM.falla_apilado > 1.5 && ~yo_arriba))
        t_ap = t_ap + dt;
    else
        t_ap = 0;
    end
    if t_ap >= 1.0
        falla = true;
    end
end
if falla && ~fh && ob.fsm >= 1 && ob.fsm <= 6
    fh = true;
    ob.fsm = 7;
    T7 = u_prev(1);
end
if tr(3) > 0.5
    ob.fsm = 9;                % E-stop: corte de motores (estado 8 -> 9 del original)
end
modo = 1;
if version > 1.5 && mx(7) > 0.5
    modo = 2;
end
otro = [mx(1); mx(2); mx(3); mx(4); mx(5); mx(6)];
ref = [ds(1) ds(2) ds(3) ds(4)];
if ob.fsm == 7
    % actitud nivelada, sin control de posición, empuje baja a 1.75 N/s
    T7 = max(T7 - 1.75*dt, 0);
    u = [T7; 0; 0; 0];
    if T7 <= 7.38
        ob.fsm = 9;
        u = zeros(4, 1);
    end
else
    [u, ob] = qd2_onboard_step(ob, tr(1), tr(2), ref, x_est, otro, QD2P, dt, modo);
end
u_prev = u;
bat = bat - dt*3.2e-4*u(1);   % descarga simple: ~0.005 V/s en hover
est = 3;
if ob.fsm >= 4 && ob.fsm <= 6
    if modo > 1.5
        est = ob.status;
    else
        est = 4;
    end
end
st = [ob.fsm; bat; est; u(1); double(err_com)];

== matlab function QD2_Sim_Dual/QDRONE 2 #2 (SIM)/PLANT (qd2_quad_plant) ==
  data: u input; x output size=[10 1]; F input; home input; QD2P parameter
function x = fcn(u, F, home, QD2P)
%#codegen
% PLANTA: qd2_quad_plant (traslación 3D, actitud y empuje de 1er orden, suelo).
persistent xs
if isempty(xs)
    xs = zeros(10, 1);
    xs(1) = home(1);
    xs(2) = home(2);
end
xs = qd2_quad_plant(xs, u, F, 0.002, QD2P.planta);
x = xs;

== matlab function QD2_Sim_Dual/DOWNWASH COUPLING/qd2_downwash (both ways) ==
  data: x1 input; F1 output size=[3 1]; x2 input; n input; F2 output size=[3 1]; QD2P parameter; QD2_SIM parameter
function [F1, F2] = fcn(x1, x2, n, QD2P, QD2_SIM)
%#codegen
% Downwash del dron de arriba sobre el de abajo (qd2_downwash) + turbulencia.
% QD2_SIM.dw_factor = downwash "real" / modelo del feedforward del MPC.
p1 = [x1(1) x1(2) x1(3)];
p2 = [x2(1) x2(2) x2(3)];
[Fa, sa] = qd2_downwash(p1, p2, QD2P.dw);
[Fb, sb] = qd2_downwash(p2, p1, QD2P.dw);
k = QD2_SIM.dw_factor;
F1 = k*(Fa + sa.*[n(1); n(2); n(3)]);
F2 = k*(Fb + sb.*[n(4); n(5); n(6)]);

== matlab function QD2_Sim_Dual/OPTITRACK (SIM, 100 Hz)/Measurement Conditioning (RSF) ==
  data: x1 input; d1 output size=[7 1]; x2 input; n input; t input; d2 output size=[7 1]; QD2_SIM parameter
function [d1, d2] = fcn(x1, x2, n, t, QD2_SIM)
%#codegen
% OptiTrack simulado: Corrected Pose Data [x y z roll pitch yaw isTracking]
% (mismo formato que Measurement Conditioning del MissionCtrl).
rp = QD2_SIM.ruido_pos; ry = QD2_SIM.ruido_yaw;
d1 = [x1(1) + rp*n(1); x1(2) + rp*n(2); x1(3) + rp*n(3); x1(7); x1(8); x1(9) + ry*n(4); 1];
d2 = [x2(1) + rp*n(5); x2(2) + rp*n(6); x2(3) + rp*n(7); x2(7); x2(8); x2(9) + ry*n(8); 1];
% pérdidas de rastreo programadas: filas [dron t1 t2]
tk = QD2_SIM.trk_off;
for i = 1:size(tk, 1)
    if t >= tk(i,2) && t < tk(i,3)
        if tk(i,1) == 1
            d1 = [nan(6,1); 0];
        elseif tk(i,1) == 2
            d2 = [nan(6,1); 0];
        end
    end
end

== matlab function QD2_Sim_Dual/SETPOINT SELECT (PID: GUARD, MPC: DIRECT) ==
  data: version input; sp1 output size=[4 1]; sp1_m input; sp2_m input; sp1_g input; sp2_g input; guard_g input; sp2 output size=[4 1]; guard output size=1
function [sp1, sp2, guard] = fcn(version, sp1_m, sp2_m, sp1_g, sp2_g, guard_g)
%#codegen
% PID: consignas del SEPARATION GUARD. MPC: consignas del supervisor (apilado
% permitido, el MPC a bordo compensa el downwash).
if version < 1.5
    sp1 = sp1_g; sp2 = sp2_g; guard = guard_g;
else
    sp1 = sp1_m; sp2 = sp2_m; guard = 0;
end
